simulink model "PID23y"  (Simulink 6.6)
settings: Solver=FixedStepDiscrete  StartTime=0.0  StopTime=10  FixedStep=0.001  RelTol=1e-3
undefined symbols (not defined in the file or in its folder): QEIInit
libraries: dsPICdrivers x12, simulink x8, dspswit3 x1, powerlib_extras x1
settings Model: Creator=123  LastModifiedBy=123  ProdHWDeviceType=16-bit Generic
settings OptimizationCC: OptimizeModelRefInitCode=on  LifeSpan=1
settings HardwareCC: ProdBitPerInt=16  ProdEndianess=LittleEndian  ProdWordSize=16  ProdHWDeviceType=16-bit Generic  TargetHWDeviceType=32-bit Generic
settings RTWCC: SystemTargetFile=dspic.tlc  TemplateMakefile=dspic_pic30_gcc.tmf  PostCodeGenCommand=dsPIC_Compile()  Description=Embedded Target for Microchip dsPIC (real-time)  ProcessScript=dspic_make_rtw_hook  CustomSource=myQEI.c
settings CodeAppCC: IgnoreCustomStorageClasses=off
settings STFCustomTargetCC: TargetFcnLib=ansi_tfl_tmw.mat  GenFloatMathFcnCalls=ANSI_C  ModelReferenceCompliant=off  IncludeMdlTerminateFcn=off  CombineOutputUpdateFcns=on  SuppressErrorStatus=on  ERTCustomFileBanners=on  SupportContinuousTime=off  SupportNonInlinedSFcns=off  SystemTargetFile=dspic.tlc
settings ERTTargetCC: TargetFcnLib=ansi_tfl_tmw.mat  GenFloatMathFcnCalls=ANSI_C  ModelReferenceCompliant=off  IncludeMdlTerminateFcn=off  SuppressErrorStatus=on  ModelStepFunctionPrototypeControlCompliant=off  InlinedParameterPlacement=NonHierarchical  ERTSrcFileBannerTemplate=dsPIC_code_template.cgt  ERTHdrFileBannerTemplate=dsPIC_code_template.cgt  ERTDataSrcFileTemplate=dsPIC_code_template.cgt  ERTDataHdrFileTemplate=dsPIC_code_template.cgt  ERTCustomFileTemplate=dsPIC_main.tlc
settings CustomProperty: DataType=string  Value=C:\PROGRA~2\MATLAB\R2007a\rtw\bin\win32\gmake
settings SimEventsCC: propLogEventsScheduled=0  propLogEventsExecuted=0  propLogDepartureEvents=0  propDisplayEventCalendar=0

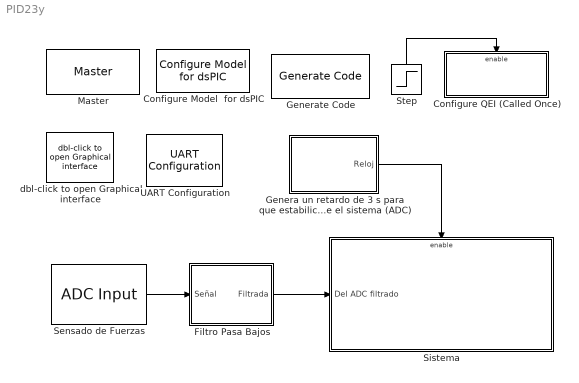
== system PID23y ==
  Configure Model  for dsPIC : dsPICdrivers/Simulink Configuration/Configure Model  for dsPIC
  Configure QEI (Called Once) : Subsystem  TreatAsAtomicUnit=on
  Filtro Pasa Bajos : Subsystem
  Genera un retardo de 3 s para que estabilice el sistema (ADC) : Subsystem
  Generate Code : dsPICdrivers/Simulink Configuration/Generate Code
  Master : dsPICdrivers/Master  Tag=dsPIC_MASTER  Priority=1  TimeStepType=Timer1  picType=30f4012  fcy=30e6  Quartz_33f=5e6  PLLActive_33f=off  fcyDesired_33f=0  tmr1="[1  29999  0]"  tmr1Info="Time Step : 0.001  ;   Error : 0%  PR1=29999"  tmr2345="[0  0  0  0]"  tmr2345cfg=[-1 -1 -1 -1]  IOautoConf=on  typePort="[ 0   0   0   0   0   0   0   0   0   0   0   0   0   0   0   0   8   0   0   0   0   0   0   0   0   0   0   0   0   0   0   0   0   0   0   0   0   0   0   0   0   0   0   0   0   0   0   0  10  10   0   0   0   0   0   0   0   0   0   0   0   0   0   0  11   0   0   0   0   0   0   0   0   0   0   0   0   0   0   0   0   0   4   5   0   0   0   0   0   0   0   0   0   0   0   0   0   0   0   0   0   0   0   0   0   0   0   0   0   0   0   0 ]"  TRIS="[ 65535  65535  65535  65532  65535  65535  65535 ]"  ADPCFG=0  MasterBusyPort=None  MasterOverloadPort=None  FOSC=FRC_PLL16  ClockSwitchMonitor=Both disabled  TempProtection_33f=TEMP_ON  FPBOR=PBOR_OFF  PWRT=PWRT_OFF  MCLR=MCLR_DIS  PowerSave=off  OverrideFcy=off  NewFcy=1e6
  Sensado de Fuerzas : dsPICdrivers/Peripheral I//O/ADC Input  Tag=dsPIC_ADC  Priority=5  ADC_TYPE=10 bits  ADC_MODE=Continuous sampling & get last channel value  NbrSampleStep=1  VoltRefpopup="AVdd  -  AVss"  OutFormatBitspopup=0000 00dd dddd dddd : Integer  InterruptPriority=1  ANCHANNELS=[0]  MaxName=ANmax = 1024  Rin=1e2  ADCS=9  SAMC=1  Temperature=25  DMAChannel=0  SampleTime=.001  Status="OK  |  Tsmp=1.667e-007 |  T/Channel=2.167e-006 |  Tall=2.167e-006"
  Sistema : Subsystem  TreatAsAtomicUnit=on
  Step : Step  Orientation=up  Time=0.002  Before=1  After=0  SampleTime=0.001
  UART Configuration : dsPICdrivers/Serial PORT/UART Configuration  Tag=dsPIC_config_UART  Priority=2  UART=1  proposed_BAUD=2400  ALT_TX_RX=off  InterruptTxWhen=When Transmit Buffer is empty  TXInterruptPri=1  TxBufferSize=32  TXEN=on  InterruptRxWhen=When Receive Buffer is full (contain 4 characters)  RXInterruptPri=2  RxBufferSize=32  BAUD=2400  UxBRG=780  Info="UxBRG = 780   ||  Real Baud : 2401   ||  % error : 0.03201  ||  max 0.24008 Bytes / Step"  RealBaud=0
  dbl-click to open Graphical interface : dsPICdrivers/Serial PORT/dbl-click to open Graphical interface  SystemSampleTime=-1  Nothing=0
  wires:
  Step/1 -> Configure QEI (Called Once)/Enable
  Genera un retardo de 3 s para que estabilice el sistema (ADC)/1(Reloj) -> Sistema/Enable
  Filtro Pasa Bajos/1(Filtrada) -> Sistema/1(Del ADC filtrado)
  Sensado de Fuerzas/1 -> Filtro Pasa Bajos/1(Señal)

== system PID23y/Configure QEI (Called Once) ==
  Enable : EnablePort
  InitQEI  (Called Once) : dsPICdrivers/OTHERS/C Function Call  Tag=dsPIC_dsPIC_CFunctionCall  fctName='QEIInit'  INPUT_SIZE=1  INPUT1=--  INPUT2=--  INPUT3=--  OUTPUT_SIZE=1  OUTPUT1=--  SampleTime=inf  InputType=[ ]  OutputType=[ ]  FctDeclaration=extern void QEIInit();  FctCall=QEIInit();  OrderingInOutPopup=None

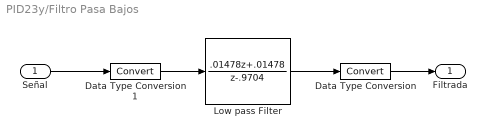
== system PID23y/Filtro Pasa Bajos ==
  Señal : Inport
  Data Type Conversion : DataTypeConversion  OutDataTypeMode=uint16  SampleTime=.001
  Data Type Conversion1 : DataTypeConversion  OutDataTypeMode=double  SampleTime=.001
  Low pass Filter : DiscreteTransferFcn  Numerator="[.01478  .01478]"  Denominator=[1 -.9704]  SampleTime=.001
  Filtrada : Outport
  wires:
  Data Type Conversion1/1 -> Low pass Filter/1
  Low pass Filter/1 -> Data Type Conversion/1
  Data Type Conversion/1 -> Filtrada/1
  Señal/1 -> Data Type Conversion1/1

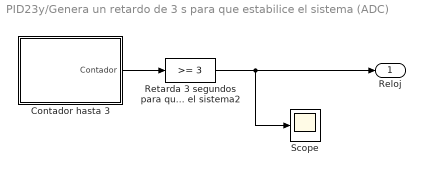
== system PID23y/Genera un retardo de 3 s para que estabilice el sistema (ADC) ==
  Contador hasta 3 : Subsystem
  Retarda 3 segundos para que estabilice el sistema2 : simulink/Logic and Bit Operations/Compare To Constant  SystemSampleTime=-1  relop=>=  const=3  LogicOutDataTypeMode=boolean  ZeroCross=off
  Scope : Scope
      settings: SaveName=ScopeData3
  Reloj : Outport
  wires:
  Contador hasta 3/1(Contador) -> Retarda 3 segundos para que estabilice el sistema2/1
  Retarda 3 segundos para que estabilice el sistema2/1 -> Reloj/1, Scope/1

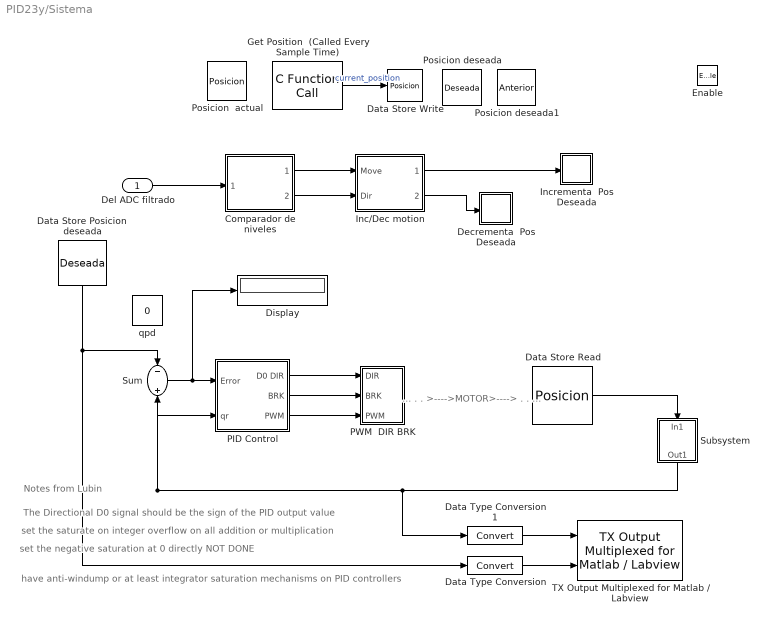
== system PID23y/Sistema ==
  note: set the saturate on integer overflow on all addition or multiplication
  note: set the negative saturation at 0 directly NOT DONE
  note: The Directional D0 signal should be the sign of the PID output value
  note: Notes from Lubin
  note: ...
      | .        .
      | >---->MOTOR>---->
      | .       .
      | ...
  note: have anti-windump or at least integrator saturation mechanisms on PID controllers
  Del ADC filtrado : Inport
  Enable : EnablePort
  Comparador de niveles : Subsystem
  Data Store Posicion  deseada : DataStoreRead  Orientation=down  DataStoreName=Deseada  SampleTime=.001
  Data Store Read : DataStoreRead  DataStoreName=Posicion  SampleTime=.001
  Data Store Write : DataStoreWrite  DataStoreName=Posicion  SampleTime=.001
  Data Type Conversion : DataTypeConversion  OutDataTypeMode=int16  SampleTime=.001
  Data Type Conversion1 : DataTypeConversion  OutDataTypeMode=int16  SampleTime=.001
  Decrementa  Pos Deseada : Subsystem  Orientation=up  TreatAsAtomicUnit=on
  Display : Display
  Get Position  (Called Every Sample Time) : dsPICdrivers/OTHERS/C Function Call  Tag=dsPIC_dsPIC_CFunctionCall  fctName='GetQEI'  INPUT_SIZE=1  INPUT1=--  INPUT2=--  INPUT3=--  OUTPUT_SIZE=1  OUTPUT1=int32  SampleTime=.001  InputType=[ ]  OutputType=[ 5 ]  FctDeclaration=extern int32_T GetQEI();  FctCall=%y1 = GetQEI();  OrderingInOutPopup=None
  Inc/Dec motion : Subsystem
  Incrementa  Pos Deseada : Subsystem  Orientation=up  TreatAsAtomicUnit=on
  PID Control : Subsystem
  PWM  DIR BRK : Subsystem
  Posicion deseada : DataStoreMemory  DataStoreName=Deseada  ReadBeforeWriteMsg=warning  WriteAfterWriteMsg=warning  WriteAfterReadMsg=warning  InitialValue=0
      settings: RTWStateStorageClass=ExportedGlobal
  Posicion deseada1 : DataStoreMemory  DataStoreName=Anterior  ReadBeforeWriteMsg=warning  WriteAfterWriteMsg=warning  WriteAfterReadMsg=warning  InitialValue=0
      settings: RTWStateStorageClass=ExportedGlobal
  Posicion  actual : DataStoreMemory  DataStoreName=Posicion  ReadBeforeWriteMsg=warning  WriteAfterWriteMsg=warning  WriteAfterReadMsg=warning  InitialValue=0
      settings: RTWStateStorageClass=ExportedGlobal
  Subsystem : Subsystem  Orientation=down
  Sum : Sum  Inputs=-+  SampleTime=.001  SaturateOnIntegerOverflow=on
  TX Output Multiplexed for Matlab / Labview : dsPICdrivers/Serial PORT/TX Output Multiplexed for Matlab // Labview  Tag=dsPIC_TX_Multiplexed  Priority=5  UART=1  CleverSpreadingChk=on  CleverSpreading=1  CHANNEL=[0 1 ]  CHANNELBLOCKED=[]  CHANNELBLOCKED_BITEWISE=0  Status=OK
  qpd : Constant  Value=0  OutDataTypeMode=int32  SampleTime=.001
  wires:
  Comparador de niveles/1(Mover) -> Inc/Dec motion/1(Move)
  Data Store Read/1 -> Subsystem/1(In1)
  Subsystem/1(Out1) -> Sum/2, PID Control/2(qr), Data Type Conversion1/1
  Sum/1 -> PID Control/1(Error), Display/1
  Comparador de niveles/2(Direccion) -> Inc/Dec motion/2(Dir)
  Inc/Dec motion/1(Increm) -> Incrementa  Pos Deseada/Enable
  Inc/Dec motion/2(Decrem) -> Decrementa  Pos Deseada/Enable
  Data Store Posicion  deseada/1 -> Data Type Conversion/1, Sum/1
  Get Position  (Called Every Sample Time)/1 -> Data Store Write/1  "current_position"
  PID Control/1(D0 DIR) -> PWM  DIR BRK/1(DIR)
  PID Control/2(BRK) -> PWM  DIR BRK/2(BRK)
  PID Control/3(" PWM") -> PWM  DIR BRK/3(PWM)
  Data Type Conversion1/1 -> TX Output Multiplexed for Matlab / Labview/1
  Data Type Conversion/1 -> TX Output Multiplexed for Matlab / Labview/2
  Del ADC filtrado/1 -> Comparador de niveles/1(Del filtro)

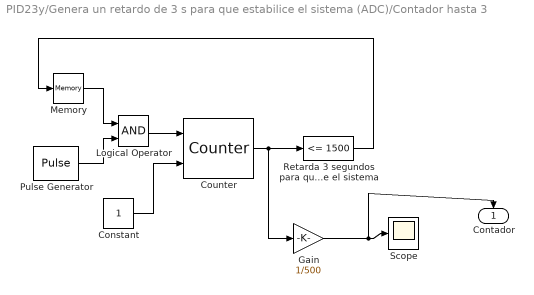
== system PID23y/Genera un retardo de 3 s para que estabilice el sistema (ADC)/Contador hasta 3 ==
  Constant : Constant
  Counter : dspswit3/Counter  Direction=Up  CountEvent=Rising edge  CounterSize=16 bits  MaxCount=255  InitialCount=0  Output=Count  HitValue=32  ResetInput=on  SamplesPerFrame=1  Ts=1  CntDtype=double  HitDtype=Logical
  Gain : Gain  Gain=1/500  SampleTime=.001
  Logical Operator : Logic  AllPortsSameDT=off  OutDataTypeMode=Boolean  SampleTime=.001
  Memory : Memory
  Pulse Generator : DiscretePulseGenerator  PulseType=Time based  Period=.002  PulseWidth=50
  Retarda 3 segundos para que estabilice el sistema : simulink/Logic and Bit Operations/Compare To Constant  SystemSampleTime=-1  relop=<=  const=1500  LogicOutDataTypeMode=boolean  ZeroCross=off
      link override Compare: Operator=>=  LogicOutDataTypeMode=Boolean  ZeroCross=off
  Scope : Scope
      settings: SaveName=ScopeData2
  Contador : Outport  Orientation=down
  wires:
  Retarda 3 segundos para que estabilice el sistema/1 -> Memory/1
  Counter/1 -> Retarda 3 segundos para que estabilice el sistema/1, Gain/1
  Logical Operator/1 -> Counter/1
  Pulse Generator/1 -> Logical Operator/2
  Memory/1 -> Logical Operator/1
  Constant/1 -> Counter/2
  Gain/1 -> Scope/1, Contador/1

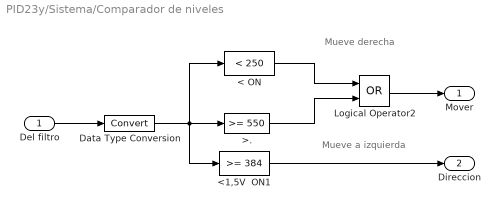
== system PID23y/Sistema/Comparador de niveles ==
  note: Mueve derecha
  note: Mueve a izquierda
  Del filtro : Inport
  < ON : simulink/Logic and Bit Operations/Compare To Constant  SystemSampleTime=-1  relop=<  const=250  LogicOutDataTypeMode=boolean  ZeroCross=off
  <1,5V  ON1 : simulink/Logic and Bit Operations/Compare To Constant  SystemSampleTime=-1  relop=>=  const=384  LogicOutDataTypeMode=boolean  ZeroCross=off
  >. : simulink/Logic and Bit Operations/Compare To Constant  SystemSampleTime=-1  relop=>=  const=550  LogicOutDataTypeMode=boolean  ZeroCross=off
  Data Type Conversion : DataTypeConversion  OutDataTypeMode=uint16  SampleTime=.001
  Logical Operator2 : Logic  Operator=OR  AllPortsSameDT=off  OutDataTypeMode=Boolean  SampleTime=.001
  Mover : Outport
  Direccion : Outport  Port=2
  wires:
  < ON/1 -> Logical Operator2/1
  >./1 -> Logical Operator2/2
  <1,5V  ON1/1 -> Direccion/1
  Logical Operator2/1 -> Mover/1
  Del filtro/1 -> Data Type Conversion/1
  Data Type Conversion/1 -> >./1, < ON/1, <1,5V  ON1/1

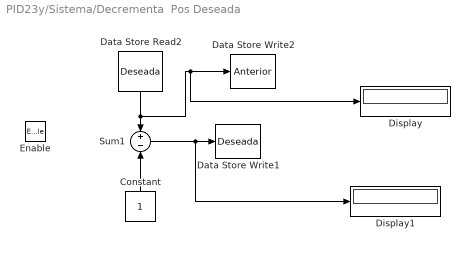
== system PID23y/Sistema/Decrementa  Pos Deseada ==
  Enable : EnablePort
  Constant : Constant  Orientation=up  OutDataTypeMode=int32  SampleTime=.001
  Data Store Read2 : DataStoreRead  Orientation=down  DataStoreName=Deseada  SampleTime=.001
  Data Store Write1 : DataStoreWrite  DataStoreName=Deseada  SampleTime=.001
  Data Store Write2 : DataStoreWrite  DataStoreName=Anterior  SampleTime=.001
  Display : Display
  Display1 : Display
  Sum1 : Sum  Inputs=+-  SampleTime=.001
  wires:
  Sum1/1 -> Data Store Write1/1, Display1/1
  Constant/1 -> Sum1/2
  Data Store Read2/1 -> Sum1/1, Data Store Write2/1, Display/1

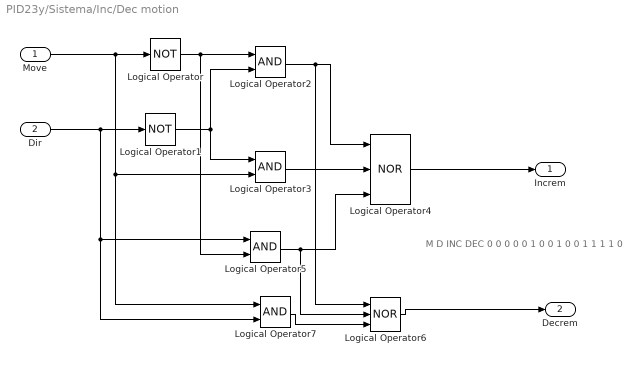
== system PID23y/Sistema/Inc/Dec motion ==
  note: M  D  INC  DEC
      | 0  0    0         0
      | 0  1    0         0
      | 1  0    0         1
      | 1  1    1         0
  Move : Inport
  Dir : Inport  Port=2
  Logical Operator : Logic  Operator=NOT  AllPortsSameDT=off  OutDataTypeMode=Boolean  SampleTime=.001
  Logical Operator1 : Logic  Operator=NOT  AllPortsSameDT=off  OutDataTypeMode=Boolean  SampleTime=.001
  Logical Operator{2..3,5,7} (4 alike) : Logic  AllPortsSameDT=off  OutDataTypeMode=Boolean  SampleTime=.001
  Logical Operator4 : Logic  Operator=NOR  Inputs=3  AllPortsSameDT=off  OutDataTypeMode=Boolean  SampleTime=.001
  Logical Operator6 : Logic  Operator=NOR  Inputs=3  AllPortsSameDT=off  OutDataTypeMode=Boolean  SampleTime=.001
  Increm : Outport
  Decrem : Outport  Port=2
  wires:
  Logical Operator4/1 -> Increm/1
  Move/1 -> Logical Operator/1, Logical Operator3/2, Logical Operator7/1
  Dir/1 -> Logical Operator1/1, Logical Operator5/1, Logical Operator7/2
  Logical Operator/1 -> Logical Operator2/1, Logical Operator5/2
  Logical Operator1/1 -> Logical Operator2/2, Logical Operator3/1
  Logical Operator2/1 -> Logical Operator4/1, Logical Operator6/1
  Logical Operator3/1 -> Logical Operator4/2
  Logical Operator5/1 -> Logical Operator4/3, Logical Operator6/2
  Logical Operator6/1 -> Decrem/1
  Logical Operator7/1 -> Logical Operator6/3

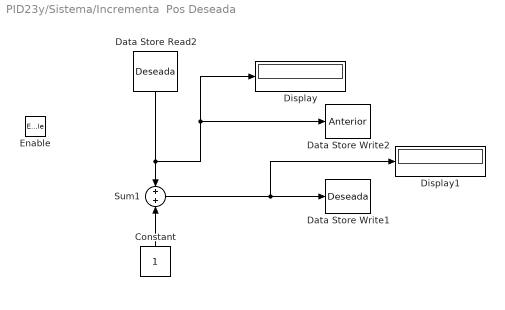
== system PID23y/Sistema/Incrementa  Pos Deseada ==
  Enable : EnablePort
  Constant : Constant  Orientation=up  OutDataTypeMode=int32  SampleTime=.001
  Data Store Read2 : DataStoreRead  Orientation=down  DataStoreName=Deseada  SampleTime=.001
  Data Store Write1 : DataStoreWrite  DataStoreName=Deseada  SampleTime=.001
  Data Store Write2 : DataStoreWrite  DataStoreName=Anterior  SampleTime=.001
  Display : Display
  Display1 : Display
  Sum1 : Sum  SampleTime=.001
  wires:
  Sum1/1 -> Data Store Write1/1, Display1/1
  Constant/1 -> Sum1/2
  Data Store Read2/1 -> Sum1/1, Data Store Write2/1, Display/1

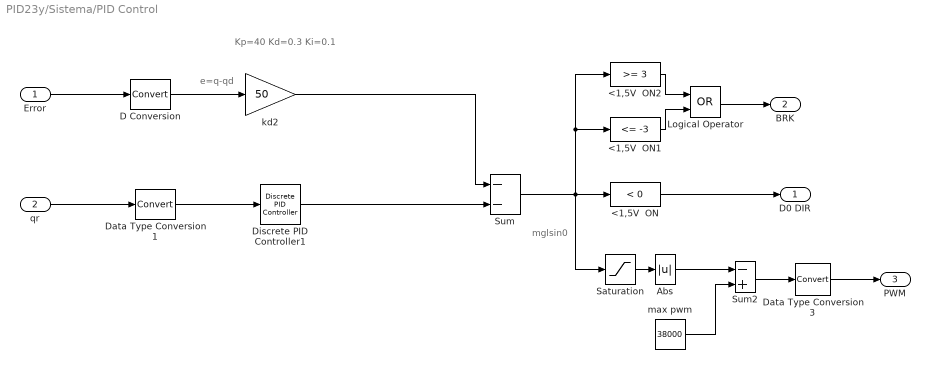
== system PID23y/Sistema/PID Control ==
  note: Kp=40
      | Kd=0.3
      | Ki=0.1
  note: e=q-qd
  note: mglsin0
  Error : Inport
  qr : Inport  Port=2
  <1,5V  ON : simulink/Logic and Bit Operations/Compare To Constant  SystemSampleTime=-1  relop=<  const=0  LogicOutDataTypeMode=boolean  ZeroCross=off
  <1,5V  ON1 : simulink/Logic and Bit Operations/Compare To Constant  SystemSampleTime=-1  relop=<=  const=-3  LogicOutDataTypeMode=boolean  ZeroCross=off
  <1,5V  ON2 : simulink/Logic and Bit Operations/Compare To Constant  SystemSampleTime=-1  relop=>=  const=3  LogicOutDataTypeMode=boolean  ZeroCross=off
  Abs : Abs  SampleTime=.001  SaturateOnIntegerOverflow=on
  D Conversion : DataTypeConversion  OutDataTypeMode=double  SampleTime=.001  SaturateOnIntegerOverflow=on
  Data Type Conversion1 : DataTypeConversion  OutDataTypeMode=double  SampleTime=.001  SaturateOnIntegerOverflow=on
  Data Type Conversion3 : DataTypeConversion  OutDataTypeMode=uint16  SampleTime=.001  SaturateOnIntegerOverflow=on
  Discrete PID Controller1 : powerlib_extras/Discrete  Control Blocks/Discrete PID Controller  DialogController=POWERSYS.PowerSysDialog  SystemSampleTime=-1  Kp=40  Ki=0.1  Kd=.3  TcD=0.5e-3  Par_Limits=[1e6 -1e6]  Init=0  Ts=.001
  Logical Operator : Logic  Operator=OR  AllPortsSameDT=off  OutDataTypeMode=Boolean  SampleTime=.001
  Saturation : Saturate  UpperLimit=38000  LowerLimit=-38000  LinearizeAsGain=off  SampleTime=.001
  Sum : Sum  Inputs=--  SampleTime=.001  SaturateOnIntegerOverflow=on
  Sum2 : Sum  Inputs=-+  SampleTime=.001  SaturateOnIntegerOverflow=on
  kd2 : Gain  Gain=50  SampleTime=.001
  max pwm : Constant  Value=38000  SampleTime=.001
  D0 DIR : Outport
  BRK : Outport  Port=2
  " PWM" : Outport  Port=3
  wires:
  Error/1 -> D Conversion/1
  Sum/1 -> <1,5V  ON/1, <1,5V  ON1/1, <1,5V  ON2/1, Saturation/1
  kd2/1 -> Sum/1
  <1,5V  ON/1 -> D0 DIR/1
  Data Type Conversion3/1 -> " PWM"/1
  D Conversion/1 -> kd2/1
  <1,5V  ON2/1 -> Logical Operator/1
  <1,5V  ON1/1 -> Logical Operator/2
  Logical Operator/1 -> BRK/1
  Saturation/1 -> Abs/1
  Data Type Conversion1/1 -> Discrete PID Controller1/1
  Discrete PID Controller1/1 -> Sum/2
  qr/1 -> Data Type Conversion1/1
  max pwm/1 -> Sum2/2
  Abs/1 -> Sum2/1
  Sum2/1 -> Data Type Conversion3/1

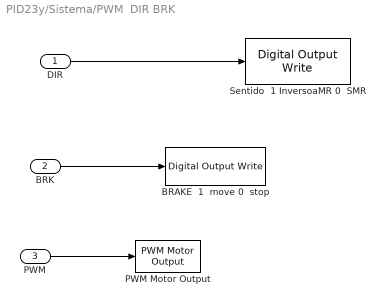
== system PID23y/Sistema/PWM  DIR BRK ==
  DIR : Inport
  BRK : Inport  Port=2
  PWM : Inport  Port=3
  BRAKE  1  move 0  stop : dsPICdrivers/Digital I//O/Digital Output Write  Tag=dsPIC_Digital_Output  Priority=5  PORT=D  Pin=[1]  Simultaneous=off  OrderingInOutPopup=None
  PWM Motor Output : dsPICdrivers/Peripheral I//O/PWM Motor Output  Tag=dsPIC_PWM_Motor  Priority=5  InputEnableChk=off  InputPeriodeChk=off  Channel=[1 ]  TPeriode=.01  PrescalerValue=16  PeriodeInteger=18750  MaxName='PWM'  Centered=off  HChannelON=off  Info="Nbr Bits : 15.1946  ||  PWM = 37500  ||  Prescaler = 16"  Delay=0  IntPriority=5  nbrPwmChannelPIC=3  Status=OK
  Sentido  1 InversoaMR 0  SMR : dsPICdrivers/Digital I//O/Digital Output Write  Tag=dsPIC_Digital_Output  Priority=5  PORT=D  Pin=[0]  Simultaneous=off  OrderingInOutPopup=None
  wires:
  DIR/1 -> Sentido  1 InversoaMR 0  SMR/1
  BRK/1 -> BRAKE  1  move 0  stop/1
  PWM/1 -> PWM Motor Output/1

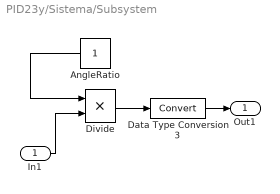
== system PID23y/Sistema/Subsystem ==
  In1 : Inport
  AngleRatio : Constant  Orientation=left  SampleTime=.001
  Data Type Conversion3 : DataTypeConversion  OutDataTypeMode=int32  SampleTime=.001
  Divide : Product  Inputs=**  OutScaling=2^-10  SampleTime=.001
  Out1 : Outport
  wires:
  AngleRatio/1 -> Divide/1
  Divide/1 -> Data Type Conversion3/1
  Data Type Conversion3/1 -> Out1/1
  In1/1 -> Divide/2
